simulink model "EV_Truck_Model"  (R2022b)
settings: Solver=FixedStepAuto  StartTime=0  StopTime=26553  FixedStep=0.1  RelTol=1e-3
model workspace (MAT data in the model file):
  ADAS_MaxAccel = 2
  ADAS_MaxDecel = 2.5
  Adas_on_off = 0
  Batt_cap_ah : Simulink.Parameter (value not decoded)
  Batt_rist_r0 : Simulink.Parameter (value not decoded)
  Batt_soc_s0 : Simulink.Parameter (value not decoded)
  Batt_volt_v0 : Simulink.Parameter (value not decoded)
  Motor_eff_100 : Simulink.Parameter (value not decoded)
  Motor_eff_190 : Simulink.Parameter (value not decoded)
  Motor_eff_95 : Simulink.Parameter (value not decoded)
  Motor_rpm_100 : Simulink.Parameter (value not decoded)
  Motor_rpm_190 : Simulink.Parameter (value not decoded)
  Motor_rpm_95 : Simulink.Parameter (value not decoded)
  Motor_torque_pos_100 : Simulink.Parameter (value not decoded)
  Motor_torque_pos_190 : Simulink.Parameter (value not decoded)
  Motor_torque_pos_95 : Simulink.Parameter (value not decoded)
  Motor_trq_190 : Simulink.Parameter (value not decoded)
  Motor_trq_95 : Simulink.Parameter (value not decoded)
  Sim_step = 0.1
  Test_DriveCycle = 0
  Trans_ratio = 6.142
  Veh_cog_fx = 1.69543
  Veh_cog_h = 0.605887
  Veh_cog_rx = 2.11956
  Veh_diff = 6.7
  Veh_whl_crr = 0.01
  Veh_whl_k = 180000
  Veh_whl_radius = 0.35
symbols that are objects in the model workspace (value not decoded): Motor_eff_100, Motor_eff_190, Motor_eff_95, Motor_rpm_100, Motor_rpm_190, Motor_rpm_95, Motor_torque_pos_100, Motor_torque_pos_190, Motor_torque_pos_95, Motor_trq_190, Motor_trq_95
undefined symbols (not defined in the file): Batt_soc_init, canChannel, Elec_aux_sw, Elec_rgn_sw, Power_option, speed, time, Veh_mass
libraries: batteryecm_lib x170, simulink x14, canmsglib x9, canlib x7, autolibshared x5, nesl_utility x4, fl_lib x3, drivingvehiclecontroller x3, hdlsllib x3, sim3dlib x1, sim3dautolib x1, vrlib x1
(part 3 of 11)

== system EV_Truck_Model/Accumulator System/Battery Pack ==
  CURR : Inport
  Controlled Current Source : fl_lib/Electrical/Electrical Sources/Controlled Current Source
  Electrical Reference : fl_lib/Electrical/Electrical Elements/Electrical Reference
  Multiply : Gain  Gain=-1
  PS-Simulink Converter : nesl_utility/PS-Simulink Converter  PhysicalDomain=network_engine_domain  SubClassName=ps_output  LeftPortType=input  RightPortType=output  PseudoPeriodic=off  Frequencies=[]  VectorFormat=inherit  Unit=inherit  AffineConversion=off
  PS-Simulink Converter1 : nesl_utility/PS-Simulink Converter  PhysicalDomain=network_engine_domain  SubClassName=ps_output  LeftPortType=input  RightPortType=output  PseudoPeriodic=off  Frequencies=[]  VectorFormat=inherit  Unit=inherit  AffineConversion=off
  SOC Terminal & Terminator : Subsystem
  Simscape HV Battery : Subsystem
      settings: PortSchema="{\"entries\":[{\"content\":{\"sides\":[{\"content\":{\"connectorIds\":[]},\"type\":\"ConnectorPlacement.EquallySpacedRectSide\",\"uuid\":\"d069fcb5-54c9-43e2-af69-b8d9e387b0b2\"},{\"content\":{\"connectorIds\":[],\"side\":\"RIGHT\"},\"type\":\"ConnectorPlacement.EquallySpacedRectSide\",\"uuid\":\"3966f711-da90-452f-b0d6-ed487d2c91a2\"},{\"content\":{\"connectorIds\":[\"LConn1\",\"LConn2\"],\"side\":\"TOP\"},\"type\":\"ConnectorPlacement.EquallySpacedRectSide\",\"uuid\":\"4ebad6b9-c403-4525-8102-5141e75b14cc\"},{\"content\":{\"connectorIds\":[\"RConn1\"],\"side\":\"BOTTOM\"},\"type\":\"ConnectorPlacement.EquallySpacedRectSide\",\"uuid\":\"0252fa9c-9f9d-4410-8a3f-59432fb9d767\"}]},\"type\":\"ConnectorPlacement.EquallySpacedConnector\",\"uuid\":\"826b9c07-966b-4c28-9a13-2c9b5485b17e\"}],\"packageUris\":[\"http://schema.mathworks.com/mf0/Connector/R2020b\"],\"version\":\"1.0\"}"
  Simulink-PS Converter : nesl_utility/Simulink-PS Converter  PhysicalDomain=network_engine_domain  SubClassName=ps_input  LeftPortType=input  RightPortType=output  PseudoPeriodic=off  Frequencies=[]  NoiseDistribution=none  NoiseParameters=[]  Unit=1  AffineConversion=off  FilteringAndDerivatives=provide  SimscapeFilterOrder=1  InputFilterTimeConstant=0.001  UdotUserProvided=0
  Solver Configuration : nesl_utility/Solver Configuration  PhysicalDomain=network_engine_domain  SubClassName=solver  LeftPortType=input  RightPortType=generic  Tones=[]  Harmonics=[]  SimulateNoise=off  Profile=off  UseLocalSampling=off  EnableSwitchedLinearOptims=on  FrequencyDomain=off  UseCCode=off  RelTol=0.001  AbsTol=0.001  MinStep=1e-09  ToWorkspace=off  RevertToSquareIcSolve=off  NumHomotopyIterations=100  PhasorMode=off  PhasorModeNumHarmonics=1  ConsistencySolver=NEWTON_XTOL_AFTER_FTOL  IndexReductionMethod=DerivativeReplacement  DoDC=off  ResidualTolerance=1e-09  ConsistencyTolSource=GLOBAL  ConsistencyAbsTol=0.001  ConsistencyRelTol=0.001  ConsistencyTolFactor=0.001  UseLocalSolver=off  LocalSolverChoice=NE_BACKWARD_EULER_ADVANCER  ResolveIndetEquations=on  FunctionEvalNumThread=1  LocalSolverSampleTime=0.001  DoFixedCost=off  MaxNonlinIter=3  MaxModeIter=2  ComputeImpulses=off  ImpulseIterations=2  LinearAlgebra=auto  LinearAlgebraNumThread=0  EquationFormulation=NE_TIME_EF  DelaysMemoryBudget=1024  AutomaticFiltering=on  FilteringTimeConstant=0.001  PartitionStorageMethod=AS_NEEDED  PartitionMemoryBudget=1024  PartitionMethod=ROBUST
  Voltage Sensor : fl_lib/Electrical/Electrical Sensors/Voltage Sensor
  VOLT : Outport
  wires:
  PS-Simulink Converter/1 -> SOC Terminal & Terminator/1(In1)
  PS-Simulink Converter1/1 -> VOLT/1  "Battery_Voltage(V)"
  CURR/1 -> Multiply/1
  Multiply/1 -> Simulink-PS Converter/1
  connections:
  Simulink-PS Converter/RConn1 -- Controlled Current Source/RConn1
  Controlled Current Source/RConn2 -- Electrical Reference/LConn1 -- Voltage Sensor/RConn2 -- Simscape HV Battery/RConn1
  Voltage Sensor/RConn1 -- PS-Simulink Converter1/LConn1
  Controlled Current Source/LConn1 -- Voltage Sensor/LConn1 -- Solver Configuration/RConn1 -- Simscape HV Battery/LConn1
  PS-Simulink Converter/LConn1 -- Simscape HV Battery/LConn2

== system EV_Truck_Model/Accumulator System/Fusible Link ==
  In1 : Inport
  Compare To Constant : simulink/Logic and Bit Operations/Compare To Constant  relop=>  const=600  OutDataTypeStr=boolean
  Compare To Constant1 : simulink/Logic and Bit Operations/Compare To Constant  relop=<  const=-600  OutDataTypeStr=boolean
  Stop Simulation : Stop
  Stop Simulation1 : Stop
  Out1 : Outport
  wires:
  Compare To Constant/1 -> Stop Simulation/1
  Compare To Constant1/1 -> Stop Simulation1/1
  In1/1 -> Out1/1, Compare To Constant1/1, Compare To Constant/1

== system EV_Truck_Model/Accumulator System/Power Calculator ==
  Current : Inport
  VOLT : Inport  Port=2
  Integrator : Integrator
  Integrator1 : Integrator
  Multiply : Gain  Gain=1/3600
  Multiply1 : Gain  Gain=1/1000
  Multiply2 : Gain  Gain=1/3600
  Product : Product
  Ampacity Consumption : Outport
  Power : Outport  Port=2
  Power Consumption : Outport  Port=3
  wires:
  Current/1 -> Product/1, Multiply/1
  Multiply/1 -> Integrator/1
  Integrator/1 -> Ampacity Consumption/1
  VOLT/1 -> Product/2
  Product/1 -> Multiply1/1
  Multiply1/1 -> Integrator1/1, Power/1
  Integrator1/1 -> Multiply2/1
  Multiply2/1 -> Power Consumption/1

== system EV_Truck_Model/Drive Cycle and Visualization/If Action Subsystem ==
  In1 : Inport
  In2 : Inport  Port=2
  Action Port : ActionPort  ActionPortLabel=if(u1 == 1)
  Constant : Constant
  Constant3 : Constant  Value=0
  Longitudinal Controller Stanley : drivingvehiclecontroller/Longitudinal Controller Stanley  Kp=2.5  Ki=1  SampleTime=Sim_step  MaxAcceleration=3.5  MaxDeceleration=4
  Saturation : Saturate  UpperLimit=100  LowerLimit=0
  Signal Specification : SignalSpecification  Unit=km/hr
  Signal Specification1 : SignalSpecification  Unit=m/s
  Terminator : Terminator
  Unit Conversion : UnitConversion
  AccelCmd : Outport
  DecelCmd : Outport  Port=2
  wires:
  Constant3/1 -> Longitudinal Controller Stanley/4
  In1/1 -> Signal Specification1/1, Longitudinal Controller Stanley/1  "DriveCycle_Speed(m/s)"
  Longitudinal Controller Stanley/2 -> DecelCmd/1
  Constant/1 -> Longitudinal Controller Stanley/3
  Longitudinal Controller Stanley/1 -> AccelCmd/1
  In2/1 -> Saturation/1
  Signal Specification1/1 -> Unit Conversion/1
  Unit Conversion/1 -> Signal Specification/1
  Signal Specification/1 -> Terminator/1  "DriveCycle_Speed(km/h)"
  Saturation/1 -> Longitudinal Controller Stanley/2

== system EV_Truck_Model/MCU and Motor System/Motor Torque Mapping and MCU Limiter ==
  TrqCmd : Inport
  Motor_RPM : Inport  Port=2
  Mux : Mux  Inputs=2
  RPM Limiter : Subsystem
  Subsystem1 : Subsystem  Commented=on
  Torque Limit Map : Subsystem
  Torque Limiter : Subsystem
  TrqLimit : Outport
  Torque : Outport  Port=2
  wires:
  Mux/1 -> TrqLimit/1
  Torque Limit Map/2(TrqLimit_min(Nm)) -> Torque Limiter/3(TrqLimit_min(Nm)), Mux/2
  Torque Limit Map/1(TrqLimit_max(Nm)) -> Torque Limiter/1(TrqLimit_max(Nm)), Mux/1
  Motor_RPM/1 -> RPM Limiter/2(RPM), Torque Limit Map/1(RPM)
  TrqCmd/1 -> Torque Limiter/2(TrqCmd)
  Torque Limiter/1(Out1) -> RPM Limiter/1(Torque)
  RPM Limiter/1(Out1) -> Torque/1

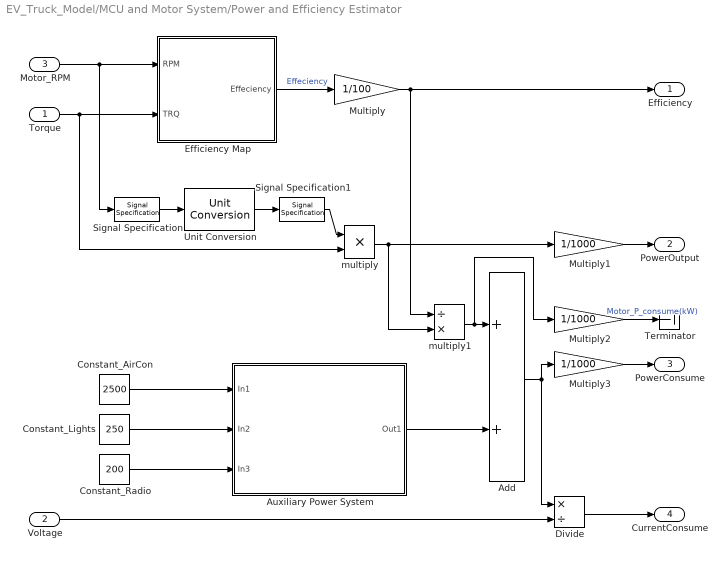
== system EV_Truck_Model/MCU and Motor System/Power and Efficiency Estimator ==
  Torque : Inport
  Voltage : Inport  Port=2
  Motor_RPM : Inport  Port=3
  Add : Sum
  Auxiliary Power System : Subsystem
  Constant_AirCon : Constant  Value=2500
  Constant_Lights : Constant  Value=250
  Constant_Radio : Constant  Value=200
  Divide : Product  Inputs=*/
  Efficiency Map : Subsystem
  Multiply : Gain  Gain=1/100
  Multiply1 : Gain  Gain=1/1000
  Multiply2 : Gain  Gain=1/1000
  Multiply3 : Gain  Gain=1/1000
  Signal Specification : SignalSpecification  Unit=rpm
  Signal Specification1 : SignalSpecification  Unit=rad/s
  Terminator : Terminator
  Unit Conversion : UnitConversion
  multiply : Product  Inputs=**
  multiply1 : Product  Inputs=/*
  Efficiency : Outport
  PowerOutput : Outport  Port=2
  PowerConsume : Outport  Port=3
  CurrentConsume : Outport  Port=4
  wires:
  Efficiency Map/1(Effeciency) -> Multiply/1  "Effeciency"
  Multiply/1 -> Efficiency/1, multiply1/1
  Torque/1 -> Efficiency Map/2(TRQ), multiply/2
  Motor_RPM/1 -> Efficiency Map/1(RPM), Signal Specification/1
  Unit Conversion/1 -> Signal Specification1/1
  multiply/1 -> multiply1/2, Multiply1/1
  Signal Specification/1 -> Unit Conversion/1
  Signal Specification1/1 -> multiply/1
  Voltage/1 -> Divide/2
  Divide/1 -> CurrentConsume/1
  Add/1 -> Divide/1, Multiply3/1
  multiply1/1 -> Multiply2/1, Add/1
  Constant_AirCon/1 -> Auxiliary Power System/1(In1)
  Constant_Lights/1 -> Auxiliary Power System/2(In2)
  Constant_Radio/1 -> Auxiliary Power System/3(In3)
  Multiply3/1 -> PowerConsume/1
  Multiply1/1 -> PowerOutput/1
  Auxiliary Power System/1(Out1) -> Add/2
  Multiply2/1 -> Terminator/1  "Motor_P_consume(kW)"

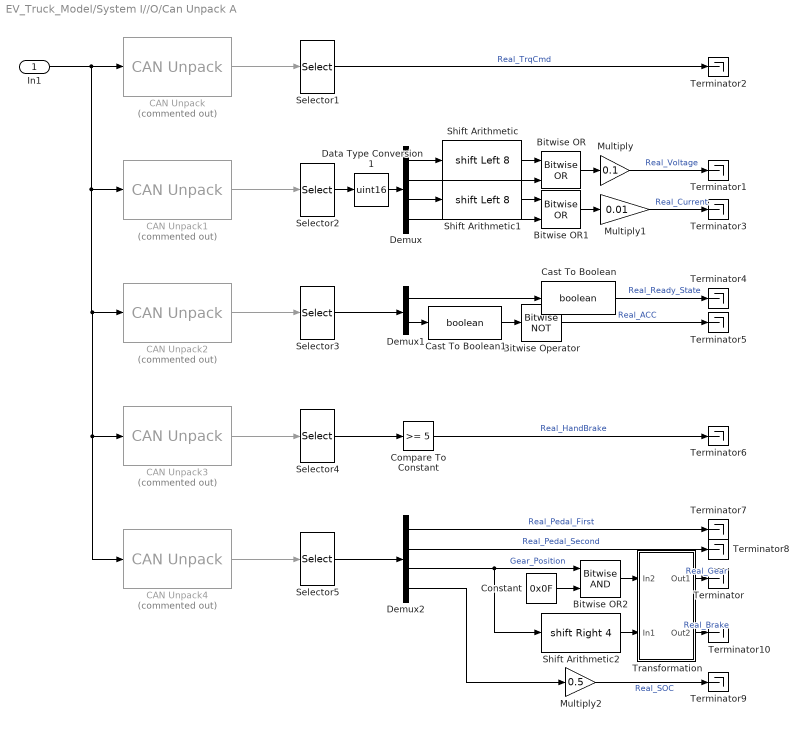
== system EV_Truck_Model/System I//O/Can Unpack A ==
  In1 : Inport
  Bitwise Operator : simulink/Logic and Bit Operations/Bitwise Operator  logicop=NOT  UseBitMask=off  BitMask=bin2dec('11011001')  BitMaskRealWorld=Stored Integer
  Bitwise OR : simulink/Logic and Bit Operations/Bitwise Operator  logicop=OR  UseBitMask=off  NumInputPorts=2  BitMask=bin2dec('11011001')  BitMaskRealWorld=Stored Integer
      settings: LibrarySourceBlock=|
      | simulink/Quick Insert/Logic and Bit
      | Operations/Bitwise AND
  Bitwise OR1 : simulink/Logic and Bit Operations/Bitwise Operator  logicop=OR  UseBitMask=off  NumInputPorts=2  BitMask=bin2dec('11011001')  BitMaskRealWorld=Stored Integer
      settings: LibrarySourceBlock=|
      | simulink/Quick Insert/Logic and Bit
      | Operations/Bitwise AND
  Bitwise OR2 : simulink/Logic and Bit Operations/Bitwise Operator  logicop=AND  UseBitMask=off  NumInputPorts=2  BitMask=bin2dec('11011001')  BitMaskRealWorld=Stored Integer
      settings: LibrarySourceBlock=|
      | simulink/Quick Insert/Logic and Bit
      | Operations/Bitwise AND
  CAN Unpack : canmsglib/CAN Unpack  Commented=on  MsgList=(none)  MsgName=CAN Msg  MsgIDType=Standard (11-bit identifier)  MsgIdentifier=0x235  MsgLength=8  SignalInfo={}  IDPort=off  TimestampPort=off  ErrorPort=off  RemotePort=off  LengthPort=off  StatusPort=off  ApplyMinMax=off
      settings: LibrarySourceBlock=embeddedtargetslib/Host Communication/CAN Unpack  DataFormat=raw data
  CAN Unpack1 : canmsglib/CAN Unpack  Commented=on  MsgList=(none)  MsgName=CAN Msg  MsgIDType=Standard (11-bit identifier)  MsgIdentifier=0x236  MsgLength=8  SignalInfo={}  IDPort=off  TimestampPort=off  ErrorPort=off  RemotePort=off  LengthPort=off  StatusPort=off  ApplyMinMax=off
      settings: LibrarySourceBlock=embeddedtargetslib/Host Communication/CAN Unpack  DataFormat=raw data
  CAN Unpack2 : canmsglib/CAN Unpack  Commented=on  MsgList=(none)  MsgName=CAN Msg  MsgIDType=Standard (11-bit identifier)  MsgIdentifier=0x338  MsgLength=8  SignalInfo={}  IDPort=off  TimestampPort=off  ErrorPort=off  RemotePort=off  LengthPort=off  StatusPort=off  ApplyMinMax=off
      settings: LibrarySourceBlock=embeddedtargetslib/Host Communication/CAN Unpack  DataFormat=raw data
  CAN Unpack3 : canmsglib/CAN Unpack  Commented=on  MsgList=(none)  MsgName=CAN Msg  MsgIDType=Standard (11-bit identifier)  MsgIdentifier=0x658  MsgLength=8  SignalInfo={}  IDPort=off  TimestampPort=off  ErrorPort=off  RemotePort=off  LengthPort=off  StatusPort=off  ApplyMinMax=off
      settings: LibrarySourceBlock=embeddedtargetslib/Host Communication/CAN Unpack  DataFormat=raw data
  CAN Unpack4 : canmsglib/CAN Unpack  Commented=on  MsgList=(none)  MsgName=CAN Msg  MsgIDType=Standard (11-bit identifier)  MsgIdentifier=0x668  MsgLength=8  SignalInfo={}  IDPort=off  TimestampPort=off  ErrorPort=off  RemotePort=off  LengthPort=off  StatusPort=off  ApplyMinMax=off
      settings: LibrarySourceBlock=embeddedtargetslib/Host Communication/CAN Unpack  DataFormat=raw data
  Cast To Boolean : DataTypeConversion  OutDataTypeStr=boolean  SaturateOnIntegerOverflow=off  RndMeth=Floor
  Cast To Boolean1 : DataTypeConversion  OutDataTypeStr=boolean  SaturateOnIntegerOverflow=off  RndMeth=Floor
  Compare To Constant : simulink/Logic and Bit Operations/Compare To Constant  relop=>=  const=5  OutDataTypeStr=boolean
  Constant : Constant  Value=0x0F
  Data Type Conversion1 : DataTypeConversion  OutDataTypeStr=uint16  SaturateOnIntegerOverflow=off  RndMeth=Floor
  Demux : Demux
  Demux1 : Demux  Outputs=2
  Demux2 : Demux
  Multiply : Gain  Gain=0.1
  Multiply1 : Gain  Gain=0.01
  Multiply2 : Gain  Gain=0.5
  Selector1 : Selector  IndexMode=Zero-based  InputPortWidth=8  IndexOptions=Index vector (dialog)  Indices=4  OutputSizes=1
  Selector2 : Selector  IndexMode=Zero-based  InputPortWidth=8  IndexOptions=Index vector (dialog)  Indices=[4 5 6 7]  OutputSizes=1
  Selector3 : Selector  IndexMode=Zero-based  InputPortWidth=8  IndexOptions=Index vector (dialog)  Indices=[6 7]  OutputSizes=1
  Selector4 : Selector  IndexMode=Zero-based  InputPortWidth=8  IndexOptions=Index vector (dialog)  Indices=7  OutputSizes=1
  Selector5 : Selector  IndexMode=Zero-based  InputPortWidth=8  IndexOptions=Index vector (dialog)  Indices=[2 3 4 7]  OutputSizes=1
  Shift Arithmetic : ArithShift  BitShiftNumber=8  BitShiftDirection=Left
  Shift Arithmetic1 : ArithShift  BitShiftNumber=8  BitShiftDirection=Left
  Shift Arithmetic2 : ArithShift  BitShiftNumber=4  BitShiftDirection=Right
  Terminator{,1..10} (11 alike) : Terminator
  Transformation : Subsystem
  wires:
  Selector1/1 -> Terminator2/1  "Real_TrqCmd"
  CAN Unpack/1 -> Selector1/1
  In1/1 -> CAN Unpack4/1, CAN Unpack3/1, CAN Unpack2/1, CAN Unpack1/1, CAN Unpack/1
  CAN Unpack1/1 -> Selector2/1
  Selector2/1 -> Data Type Conversion1/1
  Demux/2 -> Bitwise OR/2
  Shift Arithmetic/1 -> Bitwise OR/1
  Bitwise OR/1 -> Multiply/1
  Multiply/1 -> Terminator1/1  "Real_Voltage"
  Demux/1 -> Shift Arithmetic/1
  Data Type Conversion1/1 -> Demux/1
  Shift Arithmetic1/1 -> Bitwise OR1/1
  Demux/4 -> Bitwise OR1/2
  Demux/3 -> Shift Arithmetic1/1
  Bitwise OR1/1 -> Multiply1/1
  Multiply1/1 -> Terminator3/1  "Real_Current"
  CAN Unpack2/1 -> Selector3/1
  Selector3/1 -> Demux1/1
  Demux1/1 -> Cast To Boolean/1
  Cast To Boolean/1 -> Terminator4/1  "Real_Ready_State"
  Demux1/2 -> Cast To Boolean1/1
  Cast To Boolean1/1 -> Bitwise Operator/1
  Bitwise Operator/1 -> Terminator5/1  "Real_ACC"
  Selector4/1 -> Compare To Constant/1
  CAN Unpack3/1 -> Selector4/1
  Compare To Constant/1 -> Terminator6/1  "Real_HandBrake"
  CAN Unpack4/1 -> Selector5/1
  Selector5/1 -> Demux2/1
  Demux2/1 -> Terminator7/1  "Real_Pedal_First"
  Demux2/2 -> Terminator8/1  "Real_Pedal_Second"
  Demux2/3 -> Shift Arithmetic2/1, Bitwise OR2/1  "Gear_Position"
  Demux2/4 -> Multiply2/1
  Multiply2/1 -> Terminator9/1  "Real_SOC"
  Constant/1 -> Bitwise OR2/2
  Bitwise OR2/1 -> Transformation/1(In2)
  Shift Arithmetic2/1 -> Transformation/2(In1)
  Transformation/1(Out1) -> Terminator/1  "Real_Gear"
  Transformation/2(Out2) -> Terminator10/1  "Real_Brake"

== system EV_Truck_Model/System I//O/Can Unpack B  ==
  In1 : Inport
  Bitwise OR : simulink/Logic and Bit Operations/Bitwise Operator  logicop=OR  UseBitMask=off  NumInputPorts=2  BitMask=bin2dec('11011001')  BitMaskRealWorld=Stored Integer
      settings: LibrarySourceBlock=|
      | simulink/Quick Insert/Logic and Bit
      | Operations/Bitwise OR
  CAN Unpack1 : canmsglib/CAN Unpack  Commented=on  MsgList=(none)  MsgName=CAN Msg  MsgIDType=Extended (29-bit identifier)  MsgIdentifier=0x18FFE699  MsgLength=8  SignalInfo={}  IDPort=off  TimestampPort=off  ErrorPort=off  RemotePort=off  LengthPort=off  StatusPort=off  ApplyMinMax=off
      settings: LibrarySourceBlock=embeddedtargetslib/Host Communication/CAN Unpack  DataFormat=raw data
  Constant : Constant  Value=15000
  Data Type Conversion1 : DataTypeConversion  OutDataTypeStr=uint16  SaturateOnIntegerOverflow=off  RndMeth=Floor
  Demux : Demux  Outputs=2
  Minus : Sum  Inputs=+-
  Selector2 : Selector  IndexMode=Zero-based  InputPortWidth=8  IndexOptions=Index vector (dialog)  Indices=[0 1]  OutputSizes=1
  Shift Arithmetic : ArithShift  BitShiftNumber=8  BitShiftDirection=Left
  Terminator1 : Terminator
  wires:
  In1/1 -> CAN Unpack1/1
  CAN Unpack1/1 -> Selector2/1
  Selector2/1 -> Data Type Conversion1/1
  Shift Arithmetic/1 -> Bitwise OR/1
  Minus/1 -> Terminator1/1  "Real_RPM"
  Demux/1 -> Shift Arithmetic/1
  Data Type Conversion1/1 -> Demux/1
  Demux/2 -> Bitwise OR/2
  Bitwise OR/1 -> Minus/1
  Constant/1 -> Minus/2

== system EV_Truck_Model/System I//O/Command MUX ==
  thro : Inport
  brko : Inport  Port=2
  thrc : Inport  Port=3
  brkc : Inport  Port=4
  Constant : Constant  Value=0
  If : If  IfExpression=u1 == 0  ElseIfExpressions=u1 == 1  ShowElse=off
  If Action Subsystem : Subsystem  TreatAsAtomicUnit=on
  If Action Subsystem1 : Subsystem  TreatAsAtomicUnit=on
  Merge : Merge
  Merge1 : Merge
  thr : Outport
  brk : Outport  Port=2
  wires:
  Constant/1 -> If/1
  Merge/1 -> thr/1
  Merge1/1 -> brk/1
  thro/1 -> If Action Subsystem/1(In1)
  brko/1 -> If Action Subsystem/2(In2)
  If/1 -> If Action Subsystem/Action
  thrc/1 -> If Action Subsystem1/1(In1)
  brkc/1 -> If Action Subsystem1/2(In2)
  If/2 -> If Action Subsystem1/Action
  If Action Subsystem/1(Out1) -> Merge/1
  If Action Subsystem1/1(Out1) -> Merge/2
  If Action Subsystem/2(Out2) -> Merge1/1
  If Action Subsystem1/2(Out2) -> Merge1/2

== system EV_Truck_Model/System I//O/Control Mode ==
  Bit Shift : hdlsllib/Logic and Bit Operations/Bit Shift  mode=Shift Left Logical  N=4
  Bit Shift1 : hdlsllib/Logic and Bit Operations/Bit Shift  mode=Shift Left Logical  N=6
  Bit Shift2 : hdlsllib/Logic and Bit Operations/Bit Shift  mode=Shift Left Logical  N=7
  Bitwise OR : simulink/Logic and Bit Operations/Bitwise Operator  logicop=OR  UseBitMask=off  NumInputPorts=4  BitMask=bin2dec('11011001')  BitMaskRealWorld=Stored Integer
      settings: LibrarySourceBlock=|
      | simulink/Quick Insert/Logic and Bit
      | Operations/Bitwise OR
  Clock : Clock
  Constant : Constant  Value=bin2dec('10')
  Constant1 : Constant  Value=bin2dec('0')
  Counter : Stateflow chart  TreatAsAtomicUnit=on
  Data Type Conversion{,1..3} (4 alike) : DataTypeConversion  OutDataTypeStr=uint16  SaturateOnIntegerOverflow=off  RndMeth=Floor
  If : If  IfExpression=u1 > 5
  If Action Subsystem : Subsystem  TreatAsAtomicUnit=on
  If Action Subsystem1 : Subsystem  TreatAsAtomicUnit=on
  Merge : Merge
  data : Outport
  wires:
  Bitwise OR/1 -> data/1
  Data Type Conversion2/1 -> Bitwise OR/2
  Data Type Conversion1/1 -> Bitwise OR/3
  Data Type Conversion3/1 -> Bitwise OR/4
  Data Type Conversion/1 -> Bitwise OR/1
  If Action Subsystem/1(Out1) -> Merge/1
  Clock/1 -> If/1
  Bit Shift1/1 -> Data Type Conversion1/1
  If Action Subsystem1/1(Out1) -> Merge/2
  Bit Shift2/1 -> Data Type Conversion3/1
  Constant1/1 -> Bit Shift1/1
  Counter/1(count) -> Data Type Conversion/1
  If/1 -> If Action Subsystem/Action
  Bit Shift/1 -> Data Type Conversion2/1
  Constant/1 -> Bit Shift/1
  Merge/1 -> Bit Shift2/1
  If/2 -> If Action Subsystem1/Action

== system EV_Truck_Model/System I//O/Controller Remap ==
  controller : Inport
  Controller Mapping : Stateflow chart  TreatAsAtomicUnit=on
  acc : Outport
  brk : Outport  Port=2
  wires:
  Controller Mapping/1(acc) -> acc/1
  Controller Mapping/2(brk) -> brk/1
  controller/1 -> Controller Mapping/1(data)

== system EV_Truck_Model/System I//O/Subsystem ==
  Add : Sum  Inputs=++++
  Cruise Enable : Constant  Value=0  SampleTime=Sim_step
  Cruise Minus : Constant  Value=0  SampleTime=Sim_step
  Cruise Plus : Constant  Value=0  SampleTime=Sim_step
  Cruise Trigger : Constant  Value=0  SampleTime=Sim_step
  Multiply4 : Gain  Gain=2^1
  Multiply5 : Gain  Gain=2^2
  Multiply6 : Gain  Gain=2^0
  Multiply7 : Gain  Gain=2^3
  Byte0 : Outport
  wires:
  Cruise Trigger/1 -> Multiply6/1
  Add/1 -> Byte0/1  "Byte0"
  Multiply6/1 -> Add/1
  Cruise Enable/1 -> Multiply4/1
  Cruise Minus/1 -> Multiply7/1
  Cruise Plus/1 -> Multiply5/1
  Multiply7/1 -> Add/4
  Multiply5/1 -> Add/3
  Multiply4/1 -> Add/2

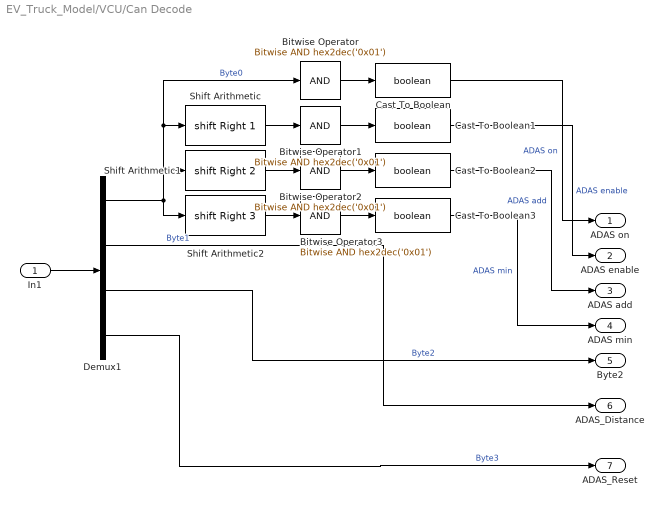
== system EV_Truck_Model/VCU/Can Decode ==
  In1 : Inport
  Bitwise Operator{,1..3} (4 alike) : simulink/Logic and Bit Operations/Bitwise Operator  logicop=AND  UseBitMask=on  BitMask=hex2dec('0x01')  BitMaskRealWorld=Stored Integer
  Cast To Boolean{,1..3} (4 alike) : DataTypeConversion  OutDataTypeStr=boolean  SaturateOnIntegerOverflow=off  RndMeth=Floor
  Demux1 : Demux
  Shift Arithmetic : ArithShift  BitShiftNumber=1  BitShiftDirection=Right
  Shift Arithmetic1 : ArithShift  BitShiftNumber=2  BitShiftDirection=Right
  Shift Arithmetic2 : ArithShift  BitShiftNumber=3  BitShiftDirection=Right
  ADAS on : Outport
  ADAS enable : Outport  Port=2
  ADAS add : Outport  Port=3
  ADAS min : Outport  Port=4
  Byte2 : Outport  Port=5
  ADAS_Distance : Outport  Port=6
  ADAS_Reset : Outport  Port=7
  wires:
  Demux1/1 -> Shift Arithmetic2/1, Bitwise Operator/1, Shift Arithmetic/1, Shift Arithmetic1/1  "Byte0"
  Shift Arithmetic/1 -> Bitwise Operator1/1
  Shift Arithmetic2/1 -> Bitwise Operator3/1
  Bitwise Operator3/1 -> Cast To Boolean3/1
  Bitwise Operator/1 -> Cast To Boolean/1
  Shift Arithmetic1/1 -> Bitwise Operator2/1
  Bitwise Operator1/1 -> Cast To Boolean1/1
  Cast To Boolean1/1 -> ADAS enable/1  "ADAS enable"
  Demux1/2 -> ADAS_Distance/1  "Byte1"
  Bitwise Operator2/1 -> Cast To Boolean2/1
  Cast To Boolean/1 -> ADAS on/1  "ADAS on"
  In1/1 -> Demux1/1
  Cast To Boolean3/1 -> ADAS min/1  "ADAS min"
  Demux1/3 -> Byte2/1  "Byte2"
  Cast To Boolean2/1 -> ADAS add/1  "ADAS add"
  Demux1/4 -> ADAS_Reset/1  "Byte3"

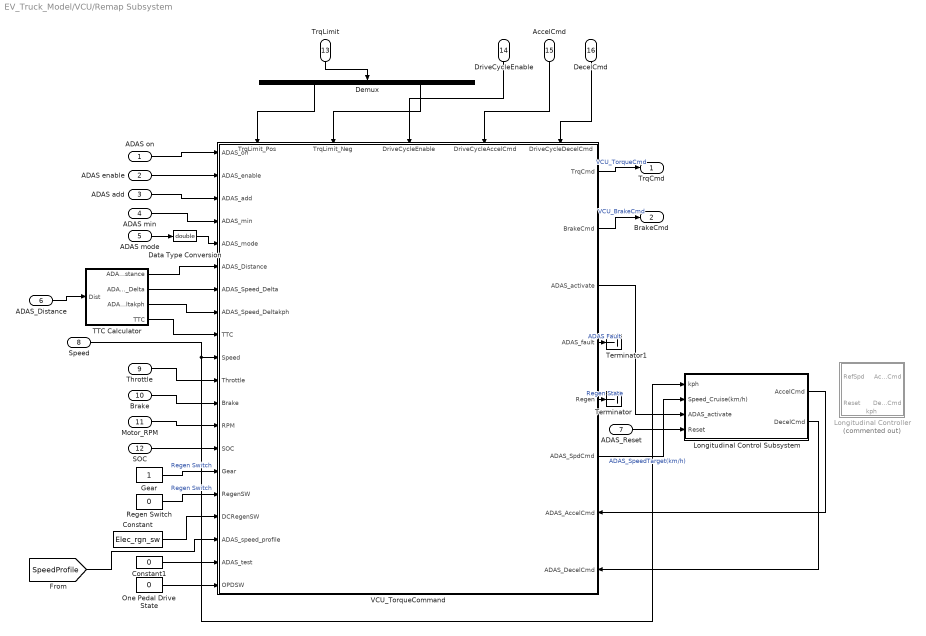
== system EV_Truck_Model/VCU/Remap Subsystem ==
  ADAS on : Inport
  ADAS enable : Inport  Port=2
  ADAS add : Inport  Port=3
  ADAS min : Inport  Port=4
  ADAS mode : Inport  Port=5
  ADAS_Distance : Inport  Port=6
  ADAS_Reset : Inport  Port=7
  Speed : Inport  Port=8
  Throttle : Inport  Port=9
  Brake : Inport  Port=10
  Motor_RPM : Inport  Port=11
  SOC : Inport  Port=12
  TrqLimit : Inport  Port=13
  DriveCycleEnable : Inport  Port=14
  AccelCmd : Inport  Port=15
  DecelCmd : Inport  Port=16
  Constant : Constant  Value=Elec_rgn_sw
  Constant1 : Constant  Value=0
  Data Type Conversion : DataTypeConversion  OutDataTypeStr=double  SaturateOnIntegerOverflow=off  RndMeth=Floor
  Demux : Demux  Outputs=2
  Gear : Constant
  Longitudinal Control Subsystem : Subsystem
  Longitudinal Controller : Subsystem  Commented=on
      settings: PortSchema="{\"entries\":[{\"content\":{\"sides\":[{\"content\":{\"connectorIds\":[\"In1\",\"In2\"]},\"type\":\"ConnectorPlacement.EquallySpacedRectSide\",\"uuid\":\"b01b53e2-4701-48b5-8c34-7fd59e654207\"},{\"content\":{\"connectorIds\":[\"Out1\",\"Out2\"],\"side\":\"RIGHT\"},\"type\":\"ConnectorPlacement.EquallySpacedRectSide\",\"uuid\":\"e91a85cf-42a7-4a33-a213-e20d411c4906\"},{\"content\":{\"connectorIds\":[],\"side\":\"TOP\"},\"type\":\"ConnectorPlacement.EquallySpacedRectSide\",\"uuid\":\"136cf3c8-ae5f-4807-b69d-541d19ec27a4\"},{\"content\":{\"connectorIds\":[\"In3\"],\"side\":\"BOTTOM\"},\"type\":\"ConnectorPlacement.EquallySpacedRectSide\",\"uuid\":\"f0fcb6e5-0d5e-4bf0-9f56-0b9b63681b2a\"}]},\"type\":\"ConnectorPlacement.EquallySpacedConnector\",\"uuid\":\"40976cb3-9931-45ff-80c5-681053a5b719\"}],\"packageUris\":[\"http://schema.mathworks.com/mf0/Connector/R2020b\"],\"version\":\"1.0\"}"
  One Pedal Drive State : Constant  Value=0
  Regen Switch : Constant  Value=0
  TTC Calculator : Subsystem
  Terminator : Terminator
  Terminator1 : Terminator
  VCU_TorqueCommand : Stateflow chart  TreatAsAtomicUnit=on
      settings: PortSchema="{\"entries\":[{\"content\":{\"sides\":[{\"content\":{\"connectorIds\":[\"In6\",\"In7\",\"In8\",\"In9\",\"In12\",\"In24\",\"In10\",\"In11\",\"In14\",\"In13\",\"In18\",\"In19\",\"In17\",\"In22\",\"In23\",\"In21\",\"In25\",\"In26\",\"In27\",\"In20\"]},\"type\":\"ConnectorPlacement.EquallySpacedRectSide\",\"uuid\":\"1e81fcdf-f4d2-4089-a69f-ddbbd6d45d8d\"},{\"content\":{\"connectorIds\":[\"Out1\",\"Out2\",\"Out3\",\"Out4\",\"Out5\",\"Out6\",\"In1\",\"In2\"],\"side\":\"RIGHT\"},\"type\":\"ConnectorPlacement.EquallySpacedRectSide\",\"uuid\":\"b926b491-4253-456a-a370-b9c8971ce6f1\"},{\"content\":{\"connectorIds\":[\"In15\",\"In16\",\"In3\",\"In4\",\"In5\"],\"side\":\"TOP\"},\"type\":\"ConnectorPlacement.EquallySpacedRectSide\",\"uuid\":\"a09473a9-286e-4628-abf4-d308fcbbd24b\"}]},\"type\":\"ConnectorPlacement.EquallySpacedConnector\",\"uuid\":\"984d4664-47bc-46a9-8fc6-7b256a69bffa\"}],\"packageUris\":[\"http://schema.mathworks.com/mf0/Connector/R2020b\"],\"version\":\"1.0\"}"
  TrqCmd : Outport
  BrakeCmd : Outport  Port=2
  wires:
  Throttle/1 -> VCU_TorqueCommand/18(Throttle)
  Brake/1 -> VCU_TorqueCommand/19(Brake)
  Regen Switch/1 -> VCU_TorqueCommand/21(RegenSW)  "Regen Switch"
  Demux/1 -> VCU_TorqueCommand/15(TrqLimit_Pos)
  Demux/2 -> VCU_TorqueCommand/16(TrqLimit_Neg)
  Motor_RPM/1 -> VCU_TorqueCommand/17(RPM)
  TrqLimit/1 -> Demux/1
  SOC/1 -> VCU_TorqueCommand/22(SOC)
  One Pedal Drive State/1 -> VCU_TorqueCommand/20(OPDSW)
  VCU_TorqueCommand/1(TrqCmd) -> TrqCmd/1  "VCU_TorqueCmd"
  VCU_TorqueCommand/2(BrakeCmd) -> BrakeCmd/1  "VCU_BrakeCmd"
  VCU_TorqueCommand/5(Regen) -> Terminator/1  "Regen State"
  Speed/1 -> Longitudinal Control Subsystem/1(kph), VCU_TorqueCommand/13(Speed)
  ADAS mode/1 -> Data Type Conversion/1
  ADAS enable/1 -> VCU_TorqueCommand/7(ADAS_enable)
  ADAS on/1 -> VCU_TorqueCommand/6(ADAS_on)
  ADAS add/1 -> VCU_TorqueCommand/8(ADAS_add)
  ADAS min/1 -> VCU_TorqueCommand/9(ADAS_min)
  Gear/1 -> VCU_TorqueCommand/23(Gear)  "Regen Switch"
  VCU_TorqueCommand/6(ADAS_SpdCmd) -> Longitudinal Control Subsystem/2(Speed_Cruise(km/h))  "ADAS_SpeedTarget(km/h)"
  VCU_TorqueCommand/3(ADAS_activate) -> Longitudinal Control Subsystem/3(ADAS_activate)
  Longitudinal Control Subsystem/1(AccelCmd) -> VCU_TorqueCommand/1(ADAS_AccelCmd)
  Longitudinal Control Subsystem/2(DecelCmd) -> VCU_TorqueCommand/2(ADAS_DecelCmd)
  TTC Calculator/1(ADAS_Distance) -> VCU_TorqueCommand/24(ADAS_Distance)
  ADAS_Distance/1 -> TTC Calculator/1(Dist)
  TTC Calculator/2(ADAS_Speed_Delta) -> VCU_TorqueCommand/10(ADAS_Speed_Delta)
  TTC Calculator/3(ADAS_Speed_Deltakph) -> VCU_TorqueCommand/11(ADAS_Speed_Deltakph)
  VCU_TorqueCommand/4(ADAS_fault) -> Terminator1/1  "ADAS Fault"
  Data Type Conversion/1 -> VCU_TorqueCommand/12(ADAS_mode)
  TTC Calculator/4(TTC) -> VCU_TorqueCommand/14(TTC)
  ADAS_Reset/1 -> Longitudinal Control Subsystem/4(Reset)
  DriveCycleEnable/1 -> VCU_TorqueCommand/3(DriveCycleEnable)
  AccelCmd/1 -> VCU_TorqueCommand/4(DriveCycleAccelCmd)
  DecelCmd/1 -> VCU_TorqueCommand/5(DriveCycleDecelCmd)
  Constant/1 -> VCU_TorqueCommand/25(DCRegenSW)
  Constant1/1 -> VCU_TorqueCommand/27(ADAS_test)
  [SpeedProfile] -> VCU_TorqueCommand/26(ADAS_speed_profile)

== system EV_Truck_Model/Vehicle Dynamics System/Driving Mileage Estimator ==
  Vehicle_Distance(km) : Inport
  SOC : Inport  Port=2
  Add : Sum  Inputs=+-
  Add1 : Sum
  Constant1 : Constant  Value=Batt_soc_init
  Divide : Product  Inputs=/*
  Product : Product
  Terminator4 : Terminator
  Terminator5 : Terminator
  wires:
  SOC/1 -> Divide/2, Add/2
  Add/1 -> Divide/1
  Divide/1 -> Product/2
  Product/1 -> Terminator4/1, Add1/2  "Vehicle_Distance_ExpLeft(km)"
  Vehicle_Distance(km)/1 -> Add1/1, Product/1
  Add1/1 -> Terminator5/1  "Vehicle_Distance_ExpTotal(km)"
  Constant1/1 -> Add/1

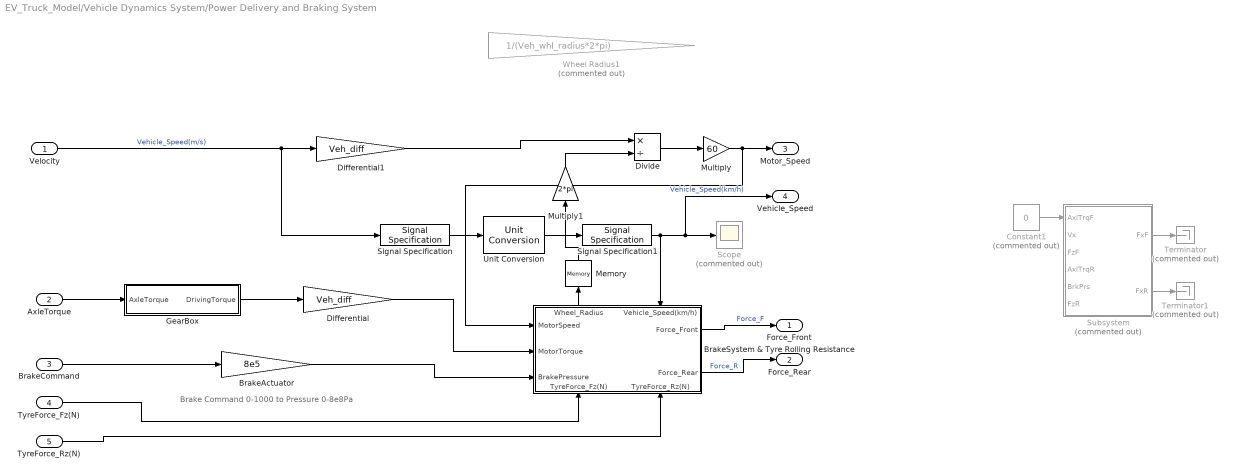
== system EV_Truck_Model/Vehicle Dynamics System/Power Delivery and Braking System ==
  note: Brake Command 0-1000 to Pressure 0-8e8Pa
  Velocity : Inport
  AxleTorque : Inport  Port=2
  BrakeCommand : Inport  Port=3
  TyreForce_Fz(N) : Inport  Port=4
  TyreForce_Rz(N) : Inport  Port=5
  BrakeActuator : Gain  Gain=8e5
  BrakeSystem & Tyre Rolling Resistance : Subsystem
      settings: PortSchema="{\"entries\":[{\"content\":{\"sides\":[{\"content\":{\"connectorIds\":[\"In1\",\"In2\",\"In3\"]},\"type\":\"ConnectorPlacement.EquallySpacedRectSide\",\"uuid\":\"c21e2244-c460-476c-838a-7bb1b56a9b61\"},{\"content\":{\"connectorIds\":[\"Out1\",\"Out2\"],\"side\":\"RIGHT\"},\"type\":\"ConnectorPlacement.EquallySpacedRectSide\",\"uuid\":\"7c7118cd-1f4a-4ad1-bba1-eac91237ebdc\"},{\"content\":{\"connectorIds\":[\"Out3\",\"In4\"],\"side\":\"TOP\"},\"type\":\"ConnectorPlacement.EquallySpacedRectSide\",\"uuid\":\"e7fdd767-540b-453b-b8c8-2862b0fff4c1\"},{\"content\":{\"connectorIds\":[\"In5\",\"In6\"],\"side\":\"BOTTOM\"},\"type\":\"ConnectorPlacement.EquallySpacedRectSide\",\"uuid\":\"66966434-46d6-405b-afe4-fca3eaeac72d\"}]},\"type\":\"ConnectorPlacement.EquallySpacedConnector\",\"uuid\":\"fa5625f8-eee5-4c95-ba72-0e5ea7a1c375\"}],\"packageUris\":[\"http://schema.mathworks.com/mf0/Connector/R2020b\"],\"version\":\"1.0\"}"
  Constant1 : Constant  Commented=on  Value=0
  Differential : Gain  Gain=Veh_diff
  Differential1 : Gain  Gain=Veh_diff
  Divide : Product  Inputs=*/
  GearBox : Subsystem
  Memory : Memory  InitialCondition=0.35
  Multiply : Gain  Gain=60
  Multiply1 : Gain  Gain=2*pi
  Scope : Scope  Commented=on
  Signal Specification : SignalSpecification
  Signal Specification1 : SignalSpecification  Unit=km/hr
  Subsystem : Subsystem  Commented=on
  Terminator : Terminator  Commented=on
  Terminator1 : Terminator  Commented=on
  Unit Conversion : UnitConversion
  Wheel Radius1 : Gain  Commented=on  Gain=1/(Veh_whl_radius*2*pi)
  Force_Front : Outport
  Force_Rear : Outport  Port=2
  Motor_Speed : Outport  Port=3
  Vehicle_Speed : Outport  Port=4
  wires:
  Velocity/1 -> Signal Specification/1, Differential1/1  "Vehicle_Speed(m/s)"
  Differential1/1 -> Divide/1
  Divide/1 -> Multiply/1
  Multiply/1 -> BrakeSystem & Tyre Rolling Resistance/1(MotorSpeed), Motor_Speed/1
  Unit Conversion/1 -> Signal Specification1/1
  Signal Specification/1 -> Unit Conversion/1
  Signal Specification1/1 -> Vehicle_Speed/1, Scope/1, BrakeSystem & Tyre Rolling Resistance/4(Vehicle_Speed(km/h))  "Vehicle_Speed(km/h)"
  Differential/1 -> BrakeSystem & Tyre Rolling Resistance/2(MotorTorque)
  BrakeCommand/1 -> BrakeActuator/1
  BrakeSystem & Tyre Rolling Resistance/2(Force_Rear) -> Force_Rear/1  "Force_R"
  BrakeActuator/1 -> BrakeSystem & Tyre Rolling Resistance/3(BrakePressure)
  Constant1/1 -> Subsystem/1(AxlTrqF)
  Subsystem/1(FxF) -> Terminator/1
  Subsystem/2(FxR) -> Terminator1/1
  BrakeSystem & Tyre Rolling Resistance/1(Force_Front) -> Force_Front/1  "Force_F"
  AxleTorque/1 -> GearBox/1(AxleTorque)
  GearBox/1(DrivingTorque) -> Differential/1
  TyreForce_Fz(N)/1 -> BrakeSystem & Tyre Rolling Resistance/5(TyreForce_Fz(N))
  TyreForce_Rz(N)/1 -> BrakeSystem & Tyre Rolling Resistance/6(TyreForce_Rz(N))
  BrakeSystem & Tyre Rolling Resistance/3(Wheel_Radius) -> Memory/1
  Multiply1/1 -> Divide/2
  Memory/1 -> Multiply1/1

== system EV_Truck_Model/Accumulator System/Battery Pack/SOC Terminal & Terminator ==
  In1 : Inport
  Compare To Constant : simulink/Logic and Bit Operations/Compare To Constant  relop=<=  const=0.001  OutDataTypeStr=boolean
  Stop Simulation : Stop
  tag scope: SOC=global
  wires:
  In1/1 -> Compare To Constant/1, [SOC]
  Compare To Constant/1 -> Stop Simulation/1

== system EV_Truck_Model/Accumulator System/Battery Pack/Simscape HV Battery ==
  Battery Semi-Pack 1 : Subsystem
  Battery Semi-Pack 2 : Subsystem
  Battery Semi-Pack 3 : Subsystem
  Battery Semi-Pack 4 : Subsystem
      settings: PortSchema="{\"entries\":[{\"content\":{\"sides\":[{\"content\":{\"connectorIds\":[\"LConn1\"]},\"type\":\"ConnectorPlacement.EquallySpacedRectSide\",\"uuid\":\"a0694fe7-d780-4483-a41f-a7ed21683973\"},{\"content\":{\"connectorIds\":[\"RConn1\"],\"side\":\"RIGHT\"},\"type\":\"ConnectorPlacement.EquallySpacedRectSide\",\"uuid\":\"39469ca5-beea-4553-8147-277bd4be0bbc\"},{\"content\":{\"connectorIds\":[\"LConn2\"],\"side\":\"TOP\"},\"type\":\"ConnectorPlacement.EquallySpacedRectSide\",\"uuid\":\"ededc17a-74df-4b2c-b94f-9a58df69fee7\"}]},\"type\":\"ConnectorPlacement.EquallySpacedConnector\",\"uuid\":\"2df81f02-ea4e-4946-bfe6-2aa0de3e9d2a\"}],\"packageUris\":[\"http://schema.mathworks.com/mf0/Connector/R2020b\"],\"version\":\"1.0\"}"
  High : PMIOPort  Side=Left
  Low : PMIOPort  Port=2  Side=Right
  SOC : PMIOPort  Port=3  Side=Left
  connections:
  Battery Semi-Pack 4/RConn1 -- Low/RConn1
  SOC/RConn1 -- Battery Semi-Pack 4/LConn2
  Battery Semi-Pack 2/LConn1 -- Battery Semi-Pack 1/RConn1
  High/RConn1 -- Battery Semi-Pack 1/LConn1
  Battery Semi-Pack 3/LConn1 -- Battery Semi-Pack 2/RConn1
  Battery Semi-Pack 4/LConn1 -- Battery Semi-Pack 3/RConn1

== system EV_Truck_Model/MCU and Motor System/Motor Torque Mapping and MCU Limiter/RPM Limiter ==
  Torque : Inport
  RPM : Inport  Port=2
  If Action Subsystem3 : Subsystem  TreatAsAtomicUnit=on
  If Action Subsystem4 : Subsystem  TreatAsAtomicUnit=on
  If1 : If  IfExpression=u1 < 4500  ElseIfExpressions=u1 > 4500  ShowElse=off
  Merge1 : Merge
  Out1 : Outport
  wires:
  If Action Subsystem4/1(Torque) -> Merge1/2
  Torque/1 -> If Action Subsystem3/1(In1), If Action Subsystem4/1(In1)
  If1/2 -> If Action Subsystem4/Action
  RPM/1 -> If Action Subsystem4/2(Motor_RPM), If1/1
  If1/1 -> If Action Subsystem3/Action
  If Action Subsystem3/1(Torque) -> Merge1/1
  Merge1/1 -> Out1/1

== system EV_Truck_Model/MCU and Motor System/Motor Torque Mapping and MCU Limiter/Subsystem1 ==
  Torque : Inport
  CurrentConsume : Inport  Port=2
  Delay : Delay  DelayLength=1
  If : If  IfExpression=u1 < 350  ElseIfExpressions=u1 >= 350  ShowElse=off
  If Action Subsystem : Subsystem  TreatAsAtomicUnit=on
  If Action Subsystem1 : Subsystem  TreatAsAtomicUnit=on
  Merge : Merge
  Out1 : Outport
  wires:
  CurrentConsume/1 -> Delay/1
  If/2 -> If Action Subsystem/Action
  If/1 -> If Action Subsystem1/Action
  Torque/1 -> If Action Subsystem1/1(Torque), If Action Subsystem/2(Torque)
  If Action Subsystem/1(Out1) -> Merge/1
  If Action Subsystem1/1(Out1) -> Merge/2
  Merge/1 -> Out1/1
  Delay/1 -> If Action Subsystem/1(CurrentConsume), If/1

== system EV_Truck_Model/MCU and Motor System/Motor Torque Mapping and MCU Limiter/Torque Limit Map ==
  RPM : Inport
  100kW Motor : Subsystem  TreatAsAtomicUnit=on
  190kW Motor : Subsystem  TreatAsAtomicUnit=on
  95kW Motor : Subsystem  TreatAsAtomicUnit=on
  Constant : Constant  Value=Power_option
  Display : Display
  Merge : Merge  Inputs=3
  Merge1 : Merge  Inputs=3
  Switch Case : SwitchCase  CaseConditions={95,132,150}  ShowDefaultCase=off
  TrqLimit_max(Nm) : Outport
  TrqLimit_min(Nm) : Outport  Port=2
  wires:
  Merge/1 -> TrqLimit_max(Nm)/1  "TrqLimit_max(Nm)"
  Merge1/1 -> TrqLimit_min(Nm)/1  "TrqLimit_min(Nm)"
  RPM/1 -> 100kW Motor/1(RPM), 95kW Motor/1(RPM), 190kW Motor/1(RPM)
  100kW Motor/1(Out1) -> Merge/1
  190kW Motor/1(Out1) -> Merge/2
  100kW Motor/2(Out2) -> Merge1/1
  190kW Motor/2(Out2) -> Merge1/2
  Constant/1 -> Display/1, Switch Case/1
  Switch Case/3 -> 190kW Motor/Action
  Switch Case/2 -> 100kW Motor/Action
  Switch Case/1 -> 95kW Motor/Action
  95kW Motor/1(Out1) -> Merge/3
  95kW Motor/2(Out2) -> Merge1/3

== system EV_Truck_Model/MCU and Motor System/Motor Torque Mapping and MCU Limiter/Torque Limiter ==
  TrqLimit_max(Nm) : Inport
  TrqCmd : Inport  Port=2
  TrqLimit_min(Nm) : Inport  Port=3
  If : If  NumInputs=3  IfExpression=u1 > u2  ElseIfExpressions=u1 < u3
  Merge : Merge  Inputs=3
  NormalTorque : Subsystem  TreatAsAtomicUnit=on
  Overtorque+ : Subsystem  TreatAsAtomicUnit=on
  Overtorque- : Subsystem  TreatAsAtomicUnit=on
  Out1 : Outport
  wires:
  TrqLimit_min(Nm)/1 -> Overtorque-/1(In1), If/3
  If/2 -> Overtorque-/Action
  TrqLimit_max(Nm)/1 -> If/2, Overtorque+/1(In1)
  Overtorque-/1(Out1) -> Merge/2
  TrqCmd/1 -> NormalTorque/1(TrqCmd), If/1
  Overtorque+/1(Out1) -> Merge/1
  If/3 -> NormalTorque/Action
  If/1 -> Overtorque+/Action
  NormalTorque/1(Out1) -> Merge/3
  Merge/1 -> Out1/1

== system EV_Truck_Model/MCU and Motor System/Power and Efficiency Estimator/Auxiliary Power System ==
  In1 : Inport
  In2 : Inport  Port=2
  In3 : Inport  Port=3
  Add : Sum  Inputs=+++
  Constant : Constant  Value=Elec_aux_sw
  If : If  IfExpression=u1 == 1
  If Action Subsystem : Subsystem  TreatAsAtomicUnit=on
  If Action Subsystem1 : Subsystem  TreatAsAtomicUnit=on
  Merge : Merge
  Out1 : Outport
  wires:
  Constant/1 -> If/1
  In1/1 -> Add/1
  In2/1 -> Add/2
  In3/1 -> Add/3
  Add/1 -> If Action Subsystem/1(In1)
  If/1 -> If Action Subsystem/Action
  If/2 -> If Action Subsystem1/Action
  If Action Subsystem1/1(Out1) -> Merge/2
  If Action Subsystem/1(Out1) -> Merge/1
  Merge/1 -> Out1/1

== system EV_Truck_Model/MCU and Motor System/Power and Efficiency Estimator/Efficiency Map ==
  RPM : Inport
  TRQ : Inport  Port=2
  100kW motor : Subsystem  TreatAsAtomicUnit=on
  190kW motor : Subsystem  TreatAsAtomicUnit=on
  95kW motor : Subsystem  TreatAsAtomicUnit=on
  Abs : Abs  SaturateOnIntegerOverflow=off
  Constant : Constant  Value=Power_option
  Merge : Merge  Inputs=3
  Switch Case : SwitchCase  CaseConditions={95,132,150}  ShowDefaultCase=off
  Effeciency : Outport
  wires:
  Abs/1 -> 95kW motor/2(TRQ POS), 190kW motor/2(TRQ POS), 100kW motor/2(TRQ POS)
  RPM/1 -> 95kW motor/1(RPM), 190kW motor/1(RPM), 100kW motor/1(RPM)
  TRQ/1 -> Abs/1
  100kW motor/1(Out1) -> Merge/3
  190kW motor/1(Out1) -> Merge/2
  Merge/1 -> Effeciency/1
  Switch Case/3 -> 190kW motor/Action
  Switch Case/2 -> 100kW motor/Action
  Constant/1 -> Switch Case/1
  Switch Case/1 -> 95kW motor/Action
  95kW motor/1(Out1) -> Merge/1

== system EV_Truck_Model/System I//O/Can Unpack A/Transformation ==
  In2 : Inport
  In1 : Inport  Port=2
  If : If  IfExpression=u1 == 4  ElseIfExpressions=u1 == 5,u1 == 6  ShowElse=off
  If Action Subsystem : Subsystem  TreatAsAtomicUnit=on
  If Action Subsystem1 : Subsystem  TreatAsAtomicUnit=on
  If Action Subsystem2 : Subsystem  TreatAsAtomicUnit=on
  If Action Subsystem3 : Subsystem  TreatAsAtomicUnit=on
  If Action Subsystem4 : Subsystem  TreatAsAtomicUnit=on
  If1 : If  IfExpression=u1 == 0  ElseIfExpressions=u1 == 1  ShowElse=off
  Merge : Merge  Inputs=3
  Merge1 : Merge
  Out1 : Outport
  Out2 : Outport  Port=2
  wires:
  In2/1 -> If/1
  If/1 -> If Action Subsystem/Action
  If/2 -> If Action Subsystem1/Action
  If/3 -> If Action Subsystem2/Action
  If Action Subsystem2/1(Out1) -> Merge/3
  If Action Subsystem1/1(Out1) -> Merge/2
  If Action Subsystem/1(Out1) -> Merge/1
  Merge/1 -> Out1/1
  In1/1 -> If1/1
  If1/1 -> If Action Subsystem3/Action
  If1/2 -> If Action Subsystem4/Action
  If Action Subsystem4/1(Out1) -> Merge1/2
  If Action Subsystem3/1(Out1) -> Merge1/1
  Merge1/1 -> Out2/1

== system EV_Truck_Model/System I//O/Command MUX/If Action Subsystem ==
  In1 : Inport
  In2 : Inport  Port=2
  Action Port : ActionPort  ActionPortLabel=if(u1 == 0)
  Out1 : Outport
  Out2 : Outport  Port=2
  wires:
  In1/1 -> Out1/1
  In2/1 -> Out2/1

== system EV_Truck_Model/System I//O/Command MUX/If Action Subsystem1 ==
  In1 : Inport
  In2 : Inport  Port=2
  Action Port : ActionPort  ActionPortLabel=elseif(u1 == 1)
  Out1 : Outport
  Out2 : Outport  Port=2
  wires:
  In1/1 -> Out1/1
  In2/1 -> Out2/1

== system EV_Truck_Model/System I//O/Control Mode/If Action Subsystem ==
  Action Port : ActionPort  ActionPortLabel=if(u1 > 5)
  Constant3 : Constant  Value=bin2dec('1')
  Out1 : Outport
  wires:
  Constant3/1 -> Out1/1

== system EV_Truck_Model/System I//O/Control Mode/If Action Subsystem1 ==
  Action Port : ActionPort  ActionPortLabel=else
  Constant2 : Constant  Value=bin2dec('0')
  Out1 : Outport
  wires:
  Constant2/1 -> Out1/1

== system EV_Truck_Model/VCU/Remap Subsystem/Longitudinal Control Subsystem ==
  kph : Inport
  Speed_Cruise(km/h) : Inport  Port=2
  ADAS_activate : Inport  Port=3
  Reset : Inport  Port=4
  Delay One Step : Delay  DelayLength=1
  Delay One Step1 : Delay  DelayLength=1
  If : If  IfExpression=u1 == 1  ShowElse=off
  If Action Subsystem : Subsystem  TreatAsAtomicUnit=on
  AccelCmd : Outport
  DecelCmd : Outport  Port=2
  wires:
  ADAS_activate/1 -> Delay One Step/1
  If/1 -> If Action Subsystem/Action
  Delay One Step/1 -> If/1
  If Action Subsystem/2(DecelCmd) -> DecelCmd/1  "ADAS_Deceleration(m/s^2)"
  If Action Subsystem/1(AccelCmd) -> AccelCmd/1  "ADAS_Acceleration(m/s^2)"
  Delay One Step1/1 -> If Action Subsystem/1(RefSpd)
  kph/1 -> If Action Subsystem/3(kph)
  Reset/1 -> If Action Subsystem/2(Reset)
  Speed_Cruise(km/h)/1 -> Delay One Step1/1

== system EV_Truck_Model/VCU/Remap Subsystem/Longitudinal Controller ==
  RefSpd : Inport
  Reset : Inport  Port=2
  kph : Inport  Port=3
  ADAS Torque Command MUX : Subsystem  Commented=on
      settings: PortSchema="{\"entries\":[{\"content\":{\"sides\":[{\"content\":{\"connectorIds\":[\"In1\",\"In2\"]},\"type\":\"ConnectorPlacement.EquallySpacedRectSide\",\"uuid\":\"6296c284-4aaa-4b65-bae8-92f6a1ca6334\"},{\"content\":{\"connectorIds\":[\"Out1\",\"Out2\"],\"side\":\"RIGHT\"},\"type\":\"ConnectorPlacement.EquallySpacedRectSide\",\"uuid\":\"12396655-9b4c-45e1-874c-981fa287baac\"},{\"content\":{\"connectorIds\":[\"In3\",\"In4\"],\"side\":\"TOP\"},\"type\":\"ConnectorPlacement.EquallySpacedRectSide\",\"uuid\":\"bc28bd2b-81fa-46c8-974f-c9b48ca64544\"}]},\"type\":\"ConnectorPlacement.EquallySpacedConnector\",\"uuid\":\"dc758841-edd4-411e-b954-73dcdfe0641a\"}],\"packageUris\":[\"http://schema.mathworks.com/mf0/Connector/R2020b\"],\"version\":\"1.0\"}"
  Constant : Constant
  Longitudinal Controller Stanley : drivingvehiclecontroller/Longitudinal Controller Stanley  Kp=2.5  Ki=1  SampleTime=0.05  MaxAcceleration=ADAS_MaxAccel  MaxDeceleration=ADAS_MaxDecel
  Memory : Memory  Commented=on
  Signal Specification : SignalSpecification  Unit=km/hr
  Signal Specification1 : SignalSpecification  Unit=m/s
  Signal Specification2 : SignalSpecification  Unit=km/hr
  Signal Specification3 : SignalSpecification  Unit=m/s
  Unit Conversion : UnitConversion
  Unit Conversion1 : UnitConversion
  Unit Delay : UnitDelay  SampleTime=-1  HasFrameUpgradeWarning=on
  Unit Delay1 : UnitDelay  SampleTime=-1  HasFrameUpgradeWarning=on
  AccelCmd : Outport
  DecelCmd : Outport  Port=2
  wires:
  Unit Conversion1/1 -> Signal Specification3/1
  Longitudinal Controller Stanley/2 -> Unit Delay/1
  Signal Specification1/1 -> Longitudinal Controller Stanley/1
  Signal Specification/1 -> Unit Conversion/1
  Signal Specification2/1 -> Unit Conversion1/1
  Longitudinal Controller Stanley/1 -> Unit Delay1/1
  Signal Specification3/1 -> Longitudinal Controller Stanley/2
  RefSpd/1 -> Signal Specification/1
  Unit Conversion/1 -> Signal Specification1/1
  Constant/1 -> Longitudinal Controller Stanley/3
  kph/1 -> Signal Specification2/1
  Unit Delay/1 -> DecelCmd/1
  Unit Delay1/1 -> AccelCmd/1
  Reset/1 -> Longitudinal Controller Stanley/4

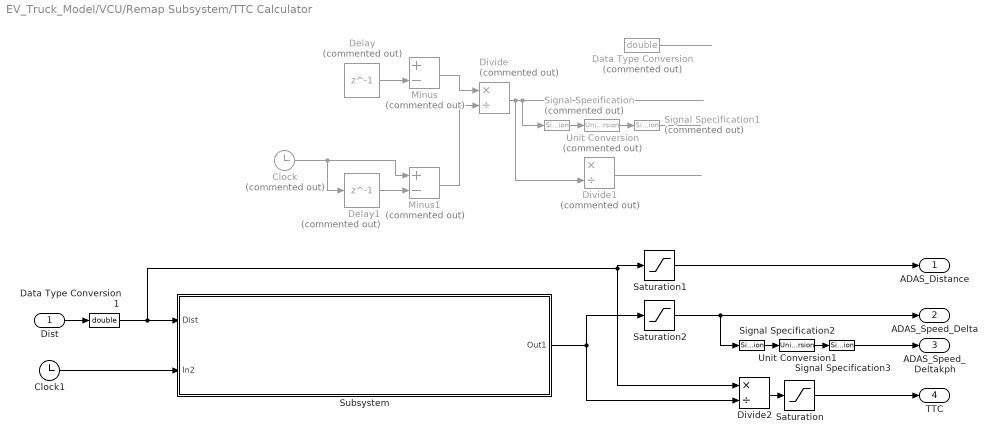
== system EV_Truck_Model/VCU/Remap Subsystem/TTC Calculator ==
  Dist : Inport
  Clock : Clock  Commented=on
  Clock1 : Clock
  Data Type Conversion : DataTypeConversion  Commented=on  OutDataTypeStr=double  SaturateOnIntegerOverflow=off  RndMeth=Floor
  Data Type Conversion1 : DataTypeConversion  OutDataTypeStr=double  SaturateOnIntegerOverflow=off  RndMeth=Floor
  Delay : Delay  Commented=on  DelayLength=1
  Delay1 : Delay  Commented=on  DelayLength=1
  Divide : Product  Commented=on  Inputs=*/
  Divide1 : Product  Commented=on  Inputs=*/
  Divide2 : Product  Inputs=*/
  Minus : Sum  Commented=on  Inputs=+-
  Minus1 : Sum  Commented=on  Inputs=+-
  Saturation : Saturate  UpperLimit=20  LowerLimit=-20
  Saturation1 : Saturate  UpperLimit=200  LowerLimit=0
  Saturation2 : Saturate  UpperLimit=10  LowerLimit=-10
  Signal Specification : SignalSpecification  Commented=on  Unit=m/s
  Signal Specification1 : SignalSpecification  Commented=on  Unit=km/hr
  Signal Specification2 : SignalSpecification  Unit=m/s
  Signal Specification3 : SignalSpecification  Unit=km/hr
  Subsystem : Subsystem
  Unit Conversion : UnitConversion  Commented=on
  Unit Conversion1 : UnitConversion
  ADAS_Distance : Outport
  ADAS_Speed_Delta : Outport  Port=2
  ADAS_Speed_Deltakph : Outport  Port=3
  TTC : Outport  Port=4
  wires:
  ? -> Delay/1, Minus/1, Divide1/1, Data Type Conversion/1
  Delay/1 -> Minus/2
  Delay1/1 -> Minus1/2
  Clock/1 -> Delay1/1, Minus1/1
  Minus/1 -> Divide/1
  Minus1/1 -> Divide/2
  Divide/1 -> Divide1/2, Signal Specification/1
  Signal Specification/1 -> Unit Conversion/1
  Unit Conversion/1 -> Signal Specification1/1
  Signal Specification1/1 -> ?
  Divide1/1 -> ?
  Data Type Conversion/1 -> ?
  Clock1/1 -> Subsystem/2(In2)
  Signal Specification2/1 -> Unit Conversion1/1
  Divide2/1 -> Saturation/1
  Saturation2/1 -> ADAS_Speed_Delta/1, Signal Specification2/1
  Subsystem/1(Out1) -> Divide2/2, Saturation2/1
  Saturation1/1 -> ADAS_Distance/1
  Saturation/1 -> TTC/1
  Unit Conversion1/1 -> Signal Specification3/1
  Signal Specification3/1 -> ADAS_Speed_Deltakph/1
  Dist/1 -> Data Type Conversion1/1
  Data Type Conversion1/1 -> Saturation1/1, Divide2/1, Subsystem/1(Dist)

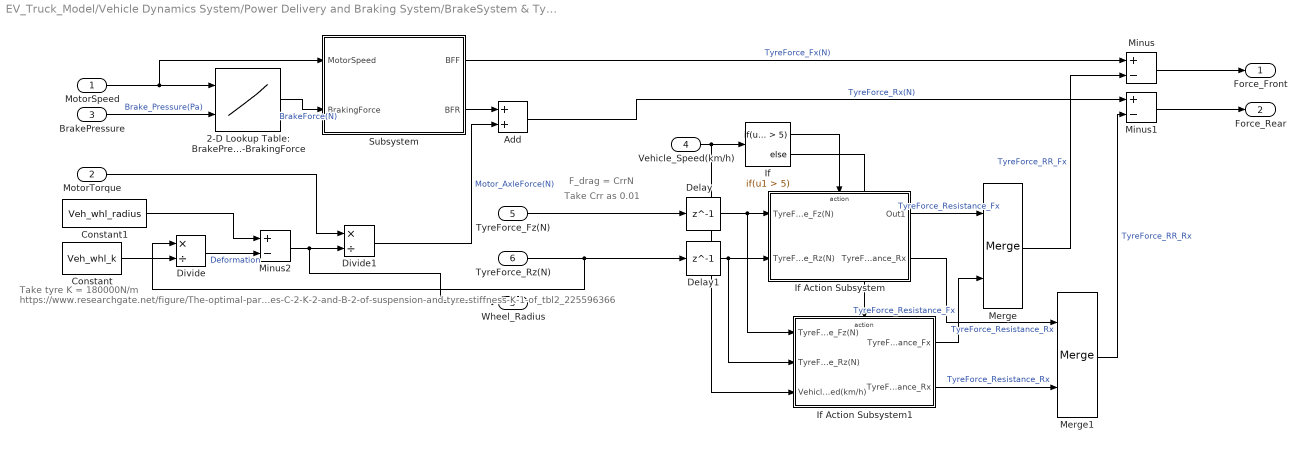
== system EV_Truck_Model/Vehicle Dynamics System/Power Delivery and Braking System/BrakeSystem & Tyre Rolling Resistance ==
  note: Take tyre K = 180000N/m
      | https://www.researchgate.net/figure/The-optimal-parameter-values-C-2-K-2-and-B-2-of-suspension-and-tyre-stiffness-K-1-of_tbl2_225596366
  note: F_drag = CrrN
  note: Take Crr as 0.01
  MotorSpeed : Inport
  MotorTorque : Inport  Port=2
  BrakePressure : Inport  Port=3
  Vehicle_Speed(km/h) : Inport  Port=4
  TyreForce_Fz(N) : Inport  Port=5
  TyreForce_Rz(N) : Inport  Port=6
  2-D Lookup Table: BrakePressure/MotorSpeed-BrakingForce : Lookup_n-D  BreakpointsForDimension1=[0;5000]  BreakpointsForDimension2=[0;1000000000]  Table=[0 32000;0 22800]  InternalRulePriority=Speed  RndMeth=Simplest
      settings: InputPortMap=u0,u1
  Add : Sum
  Constant : Constant  Value=Veh_whl_k
  Constant1 : Constant  Value=Veh_whl_radius
  Delay : Delay  DelayLength=1
  Delay1 : Delay  DelayLength=1
  Divide : Product  Inputs=*/
  Divide1 : Product  Inputs=*/
  If : If  IfExpression=u1 > 5
  If Action Subsystem : Subsystem  TreatAsAtomicUnit=on
  If Action Subsystem1 : Subsystem  TreatAsAtomicUnit=on
  Merge : Merge
  Merge1 : Merge
  Minus : Sum  Inputs=+-
  Minus1 : Sum  Inputs=+-
  Minus2 : Sum  Inputs=+-
  Subsystem : Subsystem
  Force_Front : Outport
  Force_Rear : Outport  Port=2
  Wheel_Radius : Outport  Port=3
  wires:
  TyreForce_Fz(N)/1 -> Delay/1
  TyreForce_Rz(N)/1 -> Divide/1, Delay1/1
  Merge/1 -> Minus/2  "TyreForce_RR_Fx"
  Merge1/1 -> Minus1/2  "TyreForce_RR_Rx"
  Minus1/1 -> Force_Rear/1
  Minus/1 -> Force_Front/1
  Vehicle_Speed(km/h)/1 -> If/1, If Action Subsystem1/3(Vehicle_Speed(km/h))
  If/1 -> If Action Subsystem/Action
  If/2 -> If Action Subsystem1/Action
  If Action Subsystem1/1(TyreForce_Resistance_Fx) -> Merge/2  "TyreForce_Resistance_Fx"
  If Action Subsystem/1(Out1) -> Merge/1  "TyreForce_Resistance_Fx"
  If Action Subsystem1/2(TyreForce_Resistance_Rx) -> Merge1/2  "TyreForce_Resistance_Rx"
  If Action Subsystem/2(TyreForce_Resistance_Rx) -> Merge1/1  "TyreForce_Resistance_Rx"
  Delay/1 -> If Action Subsystem1/1(TyreForce_Fz(N)), If Action Subsystem/1(TyreForce_Fz(N))
  Delay1/1 -> If Action Subsystem1/2(TyreForce_Rz(N)), If Action Subsystem/2(TyreForce_Rz(N))
  Add/1 -> Minus1/1  "TyreForce_Rx(N)"
  Subsystem/1(BFF) -> Minus/1  "TyreForce_Fx(N)"
  MotorSpeed/1 -> Subsystem/1(MotorSpeed), 2-D Lookup Table: BrakePressure/MotorSpeed-BrakingForce/1
  Divide1/1 -> Add/2  "Motor_AxleForce(N)"
  Subsystem/2(BFR) -> Add/1
  2-D Lookup Table: BrakePressure/MotorSpeed-BrakingForce/1 -> Subsystem/2(BrakingForce)  "BrakeForce(N)"
  BrakePressure/1 -> 2-D Lookup Table: BrakePressure/MotorSpeed-BrakingForce/2  "Brake_Pressure(Pa)"
  MotorTorque/1 -> Divide1/1
  Constant/1 -> Divide/2
  Constant1/1 -> Minus2/1
  Divide/1 -> Minus2/2  "Deformation"
  Minus2/1 -> Wheel_Radius/1, Divide1/2
